simulink model "UAV_controllerMCU_USBkit"  (Simulink 7.0)
settings: Solver=FixedStepDiscrete  SolverMode=SingleTasking  StartTime=0.0  StopTime=10.0  FixedStep=0.01  RelTol=1e-3
undefined symbols (not defined in the file or in its folder): IC1max, IC2max, IC3max, IC4max
libraries: dsPICdrivers x12, simulink x7
settings Model: Creator=Admin  LastModifiedBy=Admin
settings OptimizationCC: OptimizeModelRefInitCode=on  LifeSpan=1
settings HardwareCC: TargetHWDeviceType=32-bit Generic
settings RTWCC: SystemTargetFile=pic32.tlc  MakeCommand=make_CreateMPLAB  TemplateMakefile=pic32_gcc.tmf  PostCodeGenCommand=dsPIC_Compile()  Description=Embedded Target for Microchip dsPIC (real-time)  ProcessScript=pic32_make_rtw_hook
settings CodeAppCC: IgnoreCustomStorageClasses=off
settings STFCustomTargetCC: GenFloatMathFcnCalls=ANSI_C  IncludeMdlTerminateFcn=off  CombineOutputUpdateFcns=on  SuppressErrorStatus=on  ERTCustomFileBanners=on  SupportContinuousTime=off  SupportNonInlinedSFcns=off  SystemTargetFile=pic32.tlc
settings ERTTargetCC: GenFloatMathFcnCalls=ANSI_C  CompOptLevelCompliant=off  IncludeMdlTerminateFcn=off  SuppressErrorStatus=on  ModelStepFunctionPrototypeControlCompliant=off  ExtModeMexFile=noextcomm  InlinedParameterPlacement=NonHierarchical  ERTSrcFileBannerTemplate=dsPIC_code_template.cgt  ERTHdrFileBannerTemplate=dsPIC_code_template.cgt  ERTDataSrcFileTemplate=dsPIC_code_template.cgt  ERTDataHdrFileTemplate=dsPIC_code_template.cgt  ERTCustomFileTemplate=dsPIC_main.tlc
settings CustomProperty: DataType=string  Value=C:\PROGRA~1\MATLAB\R2007b\bin\win32\gmake

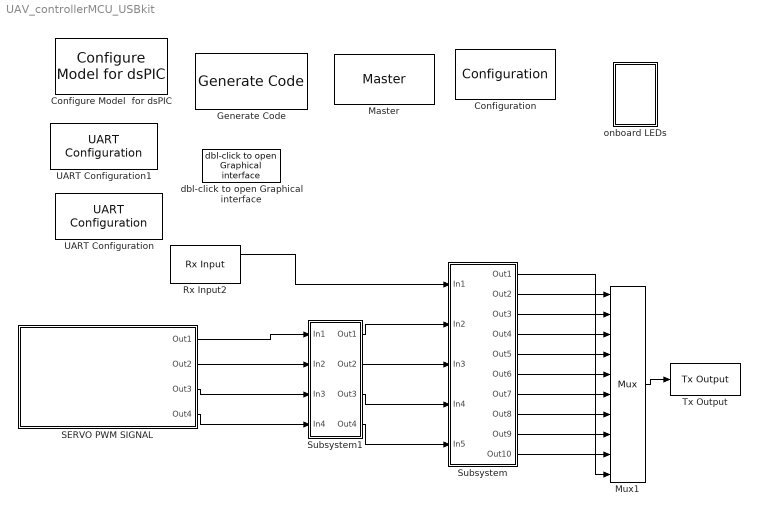
== system UAV_controllerMCU_USBkit ==
  Configuration : dsPICdrivers/Configuration  SystemSampleTime=-1  double64=off
  Configure Model  for dsPIC : dsPICdrivers/Simulink Configuration/Configure Model  for dsPIC
  Generate Code : dsPICdrivers/Simulink Configuration/Generate Code
  Master : dsPICdrivers/Master  Tag=dsPIC_MASTER  Priority=1  TimeStepType=Timer1  picType=32MX795F512L  fcy=80000000  Quartz_33f=8e6  PLLActive_33f=on  fcyDesired_33f=80e6  tmr1="[64  12499  0]"  tmr1Info="Time Step : 0.01  ;   Error : 0%  PR1=12499"  tmr2345="[8  0  0  0]"  tmr2345cfg=[-1 -1 -1 -1]  IOautoConf=on  typePort="[ 0   0   0   0   0   0   0   0   0   0   0   0   0   0   0   0   0   0   0   0   0   0   0   0   0   0   0   0   0   0   0   0   0   0   0   0   0   0   0   0   0   0   0   0   0   0   0   0  10   0  10   0   0   0   0   0   6   6   6   6   0   0   0   0   0   0   0   0   0   0   0   0   0   0   0   0   0   0   0   0   0   0   0   0   0   0   0   0   0   0   0   0   0   0   0   0   0   0   0   0   0   0   0   0   0   0   0   0   0   0   0   0 ]"  TRIS="[ 65535  65535  65535  65530  65535  65535  65535 ]"  ADPCFG=0  MasterBusyPort=None  MasterOverloadPort=None  FOSC=Quartz (XT - HS)  ClockSwitchMonitor=Both disabled  TempProtection_33f=TEMP_ON  FPBOR=<empty>  PWRT=disable  MCLR=<empty>  ICD=ICS_PGD1  JTAGEN=JTAGEN_OFF  PowerSave=off  OverrideFcy=off  NewFcy=1e6  PR2345="[65535  65535  65535  65535]"
  Mux1 : Mux  Inputs=10
  Rx Input2 : dsPICdrivers/Serial PORT/Rx Input  Tag=dsPIC_RX  Priority=5  UART=1A  SampleTime=.01  BlockingFctChk=off  OutputDefault=0  IsPresentFlagChk=on  OrderingInOutPopup=None
  SERVO PWM SIGNAL : Subsystem
  Subsystem : Subsystem
  Subsystem1 : Subsystem
  Tx Output : dsPICdrivers/Serial PORT/Tx Output  Tag=dsPIC_TX  Priority=5  UART=2A  OrderingInOutPopup=None
  UART Configuration : dsPICdrivers/Serial PORT/UART Configuration  Tag=dsPIC_config_UART  Priority=2  UART=2A  proposed_BAUD=57600  BAUD=57600  ALT_TX_RX=on  InterruptTxWhen=When Transmit Buffer is empty  TXInterruptPri=1  TxBufferSize=128  TXEN=on  InterruptRxWhen=When Receive Buffer is full (contain 4 characters)  RXInterruptPri=1  RxBufferSize=32  DoNotImplementRxInterrupt=off  DoNotImplementTxInterrupt=off  UxBRG=86  Info="UxBRG = 86   ||  Real Baud : 57471   ||  % error : -0.2235  ||  max 57.4713 Bytes / Step"  RealBaud=0  ERROR=-0.2235  BYTES_STEP=57.4713
  UART Configuration1 : dsPICdrivers/Serial PORT/UART Configuration  Tag=dsPIC_config_UART  Priority=2  UART=1A  proposed_BAUD=57600  BAUD=57600  ALT_TX_RX=on  InterruptTxWhen=When Transmit Buffer is empty  TXInterruptPri=1  TxBufferSize=128  TXEN=off  InterruptRxWhen=Do not use interrupt  RXInterruptPri=1  RxBufferSize=32  DoNotImplementRxInterrupt=off  DoNotImplementTxInterrupt=off  UxBRG=86  Info="UxBRG = 86   ||  Real Baud : 57471   ||  % error : -0.2235  ||  max 57.4713 Bytes / Step"  RealBaud=0  ERROR=-0.2235  BYTES_STEP=57.4713
  dbl-click to open Graphical interface : dsPICdrivers/Serial PORT/dbl-click to open Graphical interface  Nothing=0
  onboard LEDs : Subsystem
  wires:
  Mux1/1 -> Tx Output/1
  SERVO PWM SIGNAL/4(Out4) -> Subsystem1/4(In4)
  SERVO PWM SIGNAL/3(Out3) -> Subsystem1/3(In3)
  SERVO PWM SIGNAL/2(Out2) -> Subsystem1/2(In2)
  SERVO PWM SIGNAL/1(Out1) -> Subsystem1/1(In1)
  Rx Input2/1 -> Subsystem/1(In1)
  Subsystem/1(Out1) -> Mux1/1
  Subsystem/2(Out2) -> Mux1/2
  Subsystem/3(Out3) -> Mux1/3
  Subsystem/4(Out4) -> Mux1/4
  Subsystem/5(Out5) -> Mux1/5
  Subsystem/6(Out6) -> Mux1/6
  Subsystem/7(Out7) -> Mux1/7
  Subsystem/8(Out8) -> Mux1/8
  Subsystem/9(Out9) -> Mux1/9
  Subsystem/10(Out10) -> Mux1/10
  Subsystem1/1(Out1) -> Subsystem/2(In2)
  Subsystem1/2(Out2) -> Subsystem/3(In3)
  Subsystem1/3(Out3) -> Subsystem/4(In4)
  Subsystem1/4(Out4) -> Subsystem/5(In5)

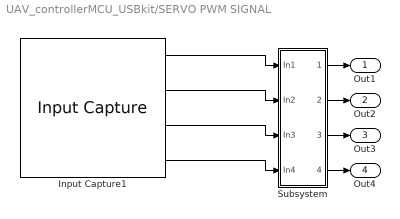
== system UAV_controllerMCU_USBkit/SERVO PWM SIGNAL ==
  Input Capture1 : dsPICdrivers/Peripheral I//O/Input Capture  Tag=dsPIC_PWM_IC  Priority=5  IntPriority=6  Channel=[ 1 2 3 4 ]  Channel_UP_Down_Periode="[1  1  1  1]"  MaxChannel="[0.001       0.001       0.001       0.001]"  SafeMarge="[10  10  10  10]"  MaxName=' IC1max , IC2max , IC3max , IC4max '  Precision="[13.2874      13.2874      13.2874      13.2874]"  Timer="[2  2  2  2]"  ChangeDetected="[0  0  0  0]"  ChangeDetectedPortRef=3  SampleTime=0.02  Status=Channel not available on selected target
  Subsystem : Subsystem
  Out1 : Outport
  Out2 : Outport  Port=2
  Out3 : Outport  Port=3
  Out4 : Outport  Port=4
  wires:
  Input Capture1/2 -> Subsystem/2(In2)
  Input Capture1/4 -> Subsystem/4(In4)
  Input Capture1/1 -> Subsystem/1(In1)
  Input Capture1/3 -> Subsystem/3(In3)
  Subsystem/1(Out1) -> Out1/1
  Subsystem/2(Out2) -> Out2/1
  Subsystem/3(Out3) -> Out3/1
  Subsystem/4(Out4) -> Out4/1

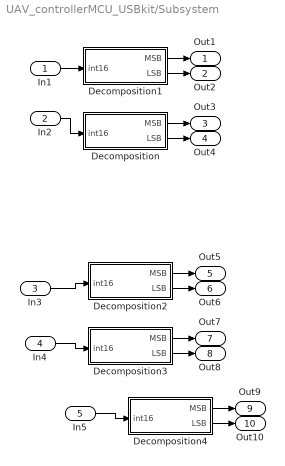
== system UAV_controllerMCU_USBkit/Subsystem ==
  In1 : Inport
  In2 : Inport  Port=2
  In3 : Inport  Port=3
  In4 : Inport  Port=4
  In5 : Inport  Port=5
  Decomposition : Subsystem
  Decomposition1 : Subsystem
  Decomposition2 : Subsystem
  Decomposition3 : Subsystem
  Decomposition4 : Subsystem
  Out1 : Outport
  Out2 : Outport  Port=2
  Out3 : Outport  Port=3
  Out4 : Outport  Port=4
  Out5 : Outport  Port=5
  Out6 : Outport  Port=6
  Out7 : Outport  Port=7
  Out8 : Outport  Port=8
  Out9 : Outport  Port=9
  Out10 : Outport  Port=10
  wires:
  In1/1 -> Decomposition1/1(int16)
  In2/1 -> Decomposition/1(int16)
  In3/1 -> Decomposition2/1(int16)
  In4/1 -> Decomposition3/1(int16)
  Decomposition1/1(MSB) -> Out1/1
  Decomposition1/2(LSB) -> Out2/1
  Decomposition/1(MSB) -> Out3/1
  Decomposition/2(LSB) -> Out4/1
  Decomposition2/1(MSB) -> Out5/1
  Decomposition2/2(LSB) -> Out6/1
  Decomposition3/1(MSB) -> Out7/1
  Decomposition3/2(LSB) -> Out8/1
  In5/1 -> Decomposition4/1(int16)
  Decomposition4/1(MSB) -> Out9/1
  Decomposition4/2(LSB) -> Out10/1

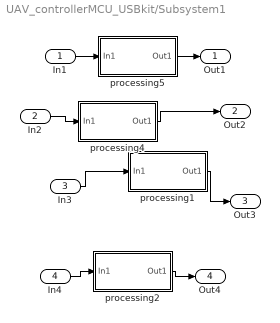
== system UAV_controllerMCU_USBkit/Subsystem1 ==
  In1 : Inport
  In2 : Inport  Port=2
  In3 : Inport  Port=3
  In4 : Inport  Port=4
  processing1 : Subsystem
  processing2 : Subsystem
  processing4 : Subsystem
  processing5 : Subsystem
  Out1 : Outport
  Out2 : Outport  Port=2
  Out3 : Outport  Port=3
  Out4 : Outport  Port=4
  wires:
  In1/1 -> processing5/1(In1)
  processing5/1(Out1) -> Out1/1
  In2/1 -> processing4/1(In1)
  processing4/1(Out1) -> Out2/1
  In3/1 -> processing1/1(In1)
  processing1/1(Out1) -> Out3/1
  In4/1 -> processing2/1(In1)
  processing2/1(Out1) -> Out4/1

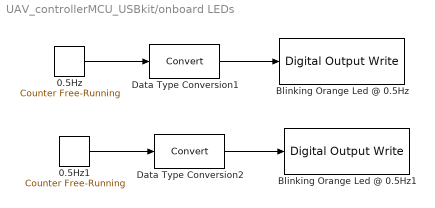
== system UAV_controllerMCU_USBkit/onboard LEDs ==
  0.5Hz : simulink/Sources/Counter Free-Running  SystemSampleTime=-1  NumBits=1  tsamp=0.02
  0.5Hz1 : simulink/Sources/Counter Free-Running  SystemSampleTime=-1  NumBits=1  tsamp=1
  Blinking Orange Led @ 0.5Hz : dsPICdrivers/Digital I//O/Digital Output Write  Tag=dsPIC_Digital_Output  Priority=5  PORT=D  Pin=[0]  Simultaneous=off  OrderingInOutPopup=None
  Blinking Orange Led @ 0.5Hz1 : dsPICdrivers/Digital I//O/Digital Output Write  Tag=dsPIC_Digital_Output  Priority=5  PORT=D  Pin=[2]  Simultaneous=off  OrderingInOutPopup=None
  Data Type Conversion1 : DataTypeConversion  OutDataTypeMode=boolean  OutDataType=sfix(16)  OutScaling=2^0
  Data Type Conversion2 : DataTypeConversion  OutDataTypeMode=boolean  OutDataType=sfix(16)  OutScaling=2^0
  wires:
  0.5Hz/1 -> Data Type Conversion1/1
  Data Type Conversion1/1 -> Blinking Orange Led @ 0.5Hz/1
  0.5Hz1/1 -> Data Type Conversion2/1
  Data Type Conversion2/1 -> Blinking Orange Led @ 0.5Hz1/1

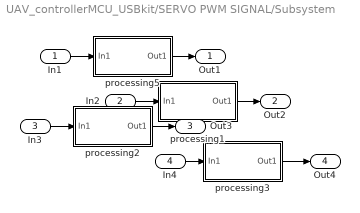
== system UAV_controllerMCU_USBkit/SERVO PWM SIGNAL/Subsystem ==
  In1 : Inport
  In2 : Inport  Port=2
  In3 : Inport  Port=3
  In4 : Inport  Port=4
  processing1 : Subsystem
  processing2 : Subsystem
  processing3 : Subsystem
  processing5 : Subsystem
  Out1 : Outport
  Out2 : Outport  Port=2
  Out3 : Outport  Port=3
  Out4 : Outport  Port=4
  wires:
  In1/1 -> processing5/1(In1)
  processing5/1(Out1) -> Out1/1
  In2/1 -> processing1/1(In1)
  processing1/1(Out1) -> Out2/1
  In3/1 -> processing2/1(In1)
  processing2/1(Out1) -> Out3/1
  In4/1 -> processing3/1(In1)
  processing3/1(Out1) -> Out4/1

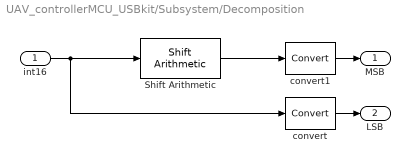
== system UAV_controllerMCU_USBkit/Subsystem/Decomposition ==
  int16 : Inport
  Shift Arithmetic : simulink/Logic and Bit Operations/Shift Arithmetic  SystemSampleTime=-1  nBitShiftRight=8  nBinPtShiftRight=0
  convert : DataTypeConversion  OutDataTypeMode=uint8  OutDataType=sfix(16)  OutScaling=2^0  ConvertRealWorld=Stored Integer (SI)
  convert1 : DataTypeConversion  OutDataTypeMode=uint8  OutDataType=sfix(16)  OutScaling=2^0  ConvertRealWorld=Stored Integer (SI)
  MSB : Outport
  LSB : Outport  Port=2
  wires:
  int16/1 -> convert/1, Shift Arithmetic/1
  Shift Arithmetic/1 -> convert1/1
  convert1/1 -> MSB/1
  convert/1 -> LSB/1

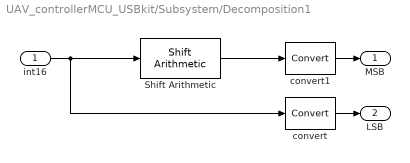
== system UAV_controllerMCU_USBkit/Subsystem/Decomposition1 ==
  int16 : Inport
  Shift Arithmetic : simulink/Logic and Bit Operations/Shift Arithmetic  SystemSampleTime=-1  nBitShiftRight=8  nBinPtShiftRight=0
  convert : DataTypeConversion  OutDataTypeMode=uint8  OutDataType=sfix(16)  OutScaling=2^0  ConvertRealWorld=Stored Integer (SI)
  convert1 : DataTypeConversion  OutDataTypeMode=uint8  OutDataType=sfix(16)  OutScaling=2^0  ConvertRealWorld=Stored Integer (SI)
  MSB : Outport
  LSB : Outport  Port=2
  wires:
  int16/1 -> convert/1, Shift Arithmetic/1
  Shift Arithmetic/1 -> convert1/1
  convert1/1 -> MSB/1
  convert/1 -> LSB/1

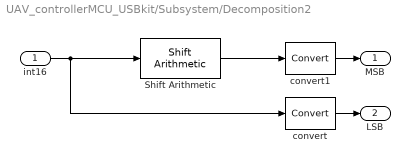
== system UAV_controllerMCU_USBkit/Subsystem/Decomposition2 ==
  int16 : Inport
  Shift Arithmetic : simulink/Logic and Bit Operations/Shift Arithmetic  SystemSampleTime=-1  nBitShiftRight=8  nBinPtShiftRight=0
  convert : DataTypeConversion  OutDataTypeMode=uint8  OutDataType=sfix(16)  OutScaling=2^0  ConvertRealWorld=Stored Integer (SI)
  convert1 : DataTypeConversion  OutDataTypeMode=uint8  OutDataType=sfix(16)  OutScaling=2^0  ConvertRealWorld=Stored Integer (SI)
  MSB : Outport
  LSB : Outport  Port=2
  wires:
  int16/1 -> convert/1, Shift Arithmetic/1
  Shift Arithmetic/1 -> convert1/1
  convert1/1 -> MSB/1
  convert/1 -> LSB/1

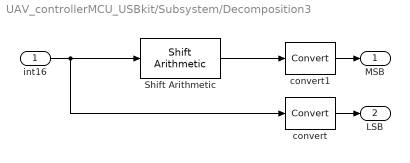
== system UAV_controllerMCU_USBkit/Subsystem/Decomposition3 ==
  int16 : Inport
  Shift Arithmetic : simulink/Logic and Bit Operations/Shift Arithmetic  SystemSampleTime=-1  nBitShiftRight=8  nBinPtShiftRight=0
  convert : DataTypeConversion  OutDataTypeMode=uint8  OutDataType=sfix(16)  OutScaling=2^0  ConvertRealWorld=Stored Integer (SI)
  convert1 : DataTypeConversion  OutDataTypeMode=uint8  OutDataType=sfix(16)  OutScaling=2^0  ConvertRealWorld=Stored Integer (SI)
  MSB : Outport
  LSB : Outport  Port=2
  wires:
  int16/1 -> convert/1, Shift Arithmetic/1
  Shift Arithmetic/1 -> convert1/1
  convert1/1 -> MSB/1
  convert/1 -> LSB/1

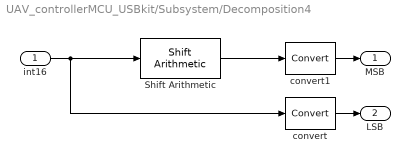
== system UAV_controllerMCU_USBkit/Subsystem/Decomposition4 ==
  int16 : Inport
  Shift Arithmetic : simulink/Logic and Bit Operations/Shift Arithmetic  SystemSampleTime=-1  nBitShiftRight=8  nBinPtShiftRight=0
  convert : DataTypeConversion  OutDataTypeMode=uint8  OutDataType=sfix(16)  OutScaling=2^0  ConvertRealWorld=Stored Integer (SI)
  convert1 : DataTypeConversion  OutDataTypeMode=uint8  OutDataType=sfix(16)  OutScaling=2^0  ConvertRealWorld=Stored Integer (SI)
  MSB : Outport
  LSB : Outport  Port=2
  wires:
  int16/1 -> convert/1, Shift Arithmetic/1
  Shift Arithmetic/1 -> convert1/1
  convert1/1 -> MSB/1
  convert/1 -> LSB/1

== system UAV_controllerMCU_USBkit/Subsystem1/processing1 ==
  In1 : Inport
  Constant : Constant  Value=IC3max/2  OutDataType=sfix(16)  OutScaling=2^0
  Data Type Conversion11 : DataTypeConversion  OutDataTypeMode=int16  OutDataType=sfix(16)  OutScaling=2^0
  Gain : Gain  Gain=10000/(0.9*IC3max)  ParameterDataType=sfix(16)  ParameterScaling=2^0  OutDataTypeMode=int16  OutDataType=sfix(16)  OutScaling=2^0
  Sum : Sum  Inputs=|+-  OutDataType=sfix(16)  OutScaling=2^0
  Out1 : Outport
  wires:
  Gain/1 -> Out1/1
  Data Type Conversion11/1 -> Sum/1
  In1/1 -> Data Type Conversion11/1
  Sum/1 -> Gain/1
  Constant/1 -> Sum/2

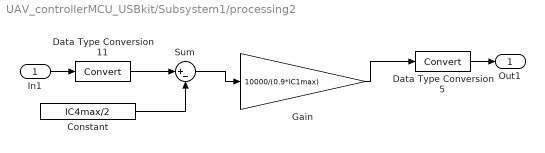
== system UAV_controllerMCU_USBkit/Subsystem1/processing2 ==
  In1 : Inport
  Constant : Constant  Value=IC4max/2  OutDataType=sfix(16)  OutScaling=2^0
  Data Type Conversion11 : DataTypeConversion  OutDataTypeMode=int16  OutDataType=sfix(16)  OutScaling=2^0
  Data Type Conversion5 : DataTypeConversion  OutDataTypeMode=int16  OutDataType=sfix(16)  OutScaling=2^0
  Gain : Gain  Gain=10000/(0.9*IC1max)  ParameterDataType=sfix(16)  ParameterScaling=2^0  OutDataTypeMode=int16  OutDataType=sfix(16)  OutScaling=2^0
  Sum : Sum  Inputs=|+-  OutDataType=sfix(16)  OutScaling=2^0
  Out1 : Outport
  wires:
  Gain/1 -> Data Type Conversion5/1
  Data Type Conversion11/1 -> Sum/1
  Data Type Conversion5/1 -> Out1/1
  In1/1 -> Data Type Conversion11/1
  Sum/1 -> Gain/1
  Constant/1 -> Sum/2

== system UAV_controllerMCU_USBkit/Subsystem1/processing4 ==
  In1 : Inport
  Constant : Constant  Value=IC2max/2  OutDataType=sfix(16)  OutScaling=2^0
  Data Type Conversion11 : DataTypeConversion  OutDataTypeMode=int16  OutDataType=sfix(16)  OutScaling=2^0
  Gain : Gain  Gain=10000/(0.9*IC2max)  ParameterDataType=sfix(16)  ParameterScaling=2^0  OutDataTypeMode=int16  OutDataType=sfix(16)  OutScaling=2^0
  Sum : Sum  Inputs=|+-  OutDataType=sfix(16)  OutScaling=2^0
  Out1 : Outport
  wires:
  Gain/1 -> Out1/1
  Data Type Conversion11/1 -> Sum/1
  In1/1 -> Data Type Conversion11/1
  Sum/1 -> Gain/1
  Constant/1 -> Sum/2

== system UAV_controllerMCU_USBkit/Subsystem1/processing5 ==
  In1 : Inport
  Constant : Constant  Value=IC1max/2  OutDataType=sfix(16)  OutScaling=2^0
  Data Type Conversion11 : DataTypeConversion  OutDataTypeMode=int16  OutDataType=sfix(16)  OutScaling=2^0
  Gain : Gain  Gain=10000/(0.9*IC1max)  ParameterDataType=sfix(16)  ParameterScaling=2^0  OutDataTypeMode=int16  OutDataType=sfix(16)  OutScaling=2^0
  Sum : Sum  Inputs=|+-  OutDataType=sfix(16)  OutScaling=2^0
  Out1 : Outport
  wires:
  Gain/1 -> Out1/1
  Data Type Conversion11/1 -> Sum/1
  In1/1 -> Data Type Conversion11/1
  Sum/1 -> Gain/1
  Constant/1 -> Sum/2

== system UAV_controllerMCU_USBkit/SERVO PWM SIGNAL/Subsystem/processing1 ==
  In1 : Inport
  Data Type Conversion11 : DataTypeConversion  OutDataTypeMode=double  OutDataType=sfix(16)  OutScaling=2^0
  Data Type Conversion5 : DataTypeConversion  OutDataTypeMode=int16  OutDataType=sfix(16)  OutScaling=2^0
  Embedded MATLAB Function1 : Stateflow chart
  Out1 : Outport
  wires:
  Embedded MATLAB Function1/1(y) -> Data Type Conversion5/1
  Data Type Conversion11/1 -> Embedded MATLAB Function1/1(u)
  Data Type Conversion5/1 -> Out1/1
  In1/1 -> Data Type Conversion11/1

== system UAV_controllerMCU_USBkit/SERVO PWM SIGNAL/Subsystem/processing2 ==
  In1 : Inport
  Data Type Conversion11 : DataTypeConversion  OutDataTypeMode=double  OutDataType=sfix(16)  OutScaling=2^0
  Data Type Conversion5 : DataTypeConversion  OutDataTypeMode=int16  OutDataType=sfix(16)  OutScaling=2^0
  Embedded MATLAB Function1 : Stateflow chart
  Out1 : Outport
  wires:
  Embedded MATLAB Function1/1(y) -> Data Type Conversion5/1
  Data Type Conversion11/1 -> Embedded MATLAB Function1/1(u)
  Data Type Conversion5/1 -> Out1/1
  In1/1 -> Data Type Conversion11/1

== system UAV_controllerMCU_USBkit/SERVO PWM SIGNAL/Subsystem/processing3 ==
  In1 : Inport
  Data Type Conversion11 : DataTypeConversion  OutDataTypeMode=double  OutDataType=sfix(16)  OutScaling=2^0
  Data Type Conversion5 : DataTypeConversion  OutDataTypeMode=int16  OutDataType=sfix(16)  OutScaling=2^0
  Embedded MATLAB Function1 : Stateflow chart
  Out1 : Outport
  wires:
  Embedded MATLAB Function1/1(y) -> Data Type Conversion5/1
  Data Type Conversion11/1 -> Embedded MATLAB Function1/1(u)
  Data Type Conversion5/1 -> Out1/1
  In1/1 -> Data Type Conversion11/1

== system UAV_controllerMCU_USBkit/SERVO PWM SIGNAL/Subsystem/processing5 ==
  In1 : Inport
  Data Type Conversion11 : DataTypeConversion  OutDataTypeMode=double  OutDataType=sfix(16)  OutScaling=2^0
  Data Type Conversion5 : DataTypeConversion  OutDataTypeMode=int16  OutDataType=sfix(16)  OutScaling=2^0
  Embedded MATLAB Function1 : Stateflow chart
  Out1 : Outport
  wires:
  Embedded MATLAB Function1/1(y) -> Data Type Conversion5/1
  Data Type Conversion11/1 -> Embedded MATLAB Function1/1(u)
  Data Type Conversion5/1 -> Out1/1
  In1/1 -> Data Type Conversion11/1

== matlab function SERVO PWM SIGNAL/Subsystem/processing3/Embedded MATLAB Function1 ==
  data: u input inherited; y output inherited
function y = fcn(u)
% This block supports the Embedded MATLAB subset.
% See the help menu for details. 
% A=3.3/2^12;
% B=1/0.0049;
B=0.015/9374;

y = 1000000*B*u;

end

== matlab function SERVO PWM SIGNAL/Subsystem/processing5/Embedded MATLAB Function1 ==
  data: u input inherited; y output inherited
function y = fcn(u)
% This block supports the Embedded MATLAB subset.
% See the help menu for details. 
% A=3.3/2^12;
% B=1/0.0049;
B=0.015/9374;

y = 1000000*B*u;

end

== matlab function SERVO PWM SIGNAL/Subsystem/processing1/Embedded MATLAB Function1 ==
  data: u input inherited; y output inherited
function y = fcn(u)
% This block supports the Embedded MATLAB subset.
% See the help menu for details. 
% A=3.3/2^12;
% B=1/0.0049;
B=0.015/9374;

y = 1000000*B*u;

end

== matlab function SERVO PWM SIGNAL/Subsystem/processing2/Embedded MATLAB Function1 ==
  data: u input inherited; y output inherited
function y = fcn(u)
% This block supports the Embedded MATLAB subset.
% See the help menu for details. 
% A=3.3/2^12;
% B=1/0.0049;
B=0.015/9374;

y = 1000000*B*u;

end
